simulink model "position_control"  (R2026a)
settings: Solver=VariableStepAuto  StopTime=3
model workspace (MAT data in the model file):
  K = Simulink.Parameter
  K.Complexity = 'real'
  K.Dimensions = [0 0]
  K.DataType = 'auto'
  Kp = Simulink.Parameter
  Kp.Complexity = 'real'
  Kp.Dimensions = [0 0]
  Kp.DataType = 'auto'
  omega_d = Simulink.Parameter
  omega_d.Complexity = 'real'
  omega_d.Dimensions = [0 0]
  omega_d.DataType = 'auto'
  sigma = Simulink.Parameter
  sigma.Complexity = 'real'
  sigma.Dimensions = [0 0]
  sigma.DataType = 'auto'
values from neighbouring files (symbols this model uses):
  K = 1.75    [Runpos_control.m]
  Kp = 2    [Runpos_control.m]
  sigma = 17.5    [Runpos_control.m]
libraries: simulink x1, slpidlib x1
settings Model: Creator=tmpad  LastModifiedBy=tmpad

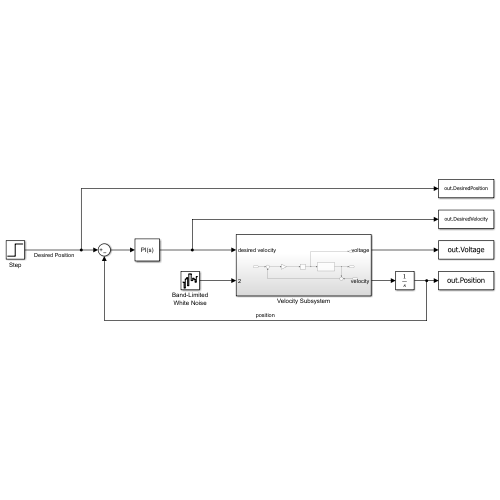
[thumbnail: Simulink's stored preview of the top-level diagram]
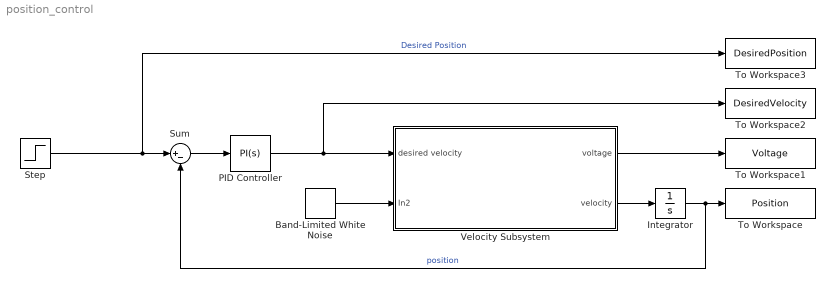
== system position_control ==
  Band-Limited White Noise : simulink/Sources/Band-Limited White Noise  Cov=[0.0001]  Ts=0.01  seed=[23341]
  Integrator : Integrator
  PID Controller : slpidlib/PID Controller  Controller=PI  Form=Parallel  TimeDomain=Continuous-time  UseExternalTs=off  SampleTime=-1  IntegratorMethod=Forward Euler  FilterMethod=Forward Euler  ControllerParametersSource=internal  P=1  I=1  UseKiTs=off  D=0  UseExternalDerivativeSource=off  N=100  UseFilter=on  TunerSelectOption=Transfer Function Based (PID Tuner App)  InitialConditionSource=internal  InitialConditionForIntegrator=0  InitialConditionForFilter=0  DifferentiatorICPrevScaledInput=0  ExternalReset=none  TrackingMode=off  Kt=1  LimitOutput=off  SatLimitsSource=internal  UpperSaturationLimit=inf  LowerSaturationLimit=-inf  LinearizeAsGain=on  AntiWindupMode=none  Kb=1  LimitIntegrator=off  UpperIntegratorSaturationLimit=inf  LowerIntegratorSaturationLimit=-inf  POutMin=[]  POutMax=[]  IOutMin=[]  IOutMax=[]  DOutMin=[]  DOutMax=[]  NOutMin=[]  NOutMax=[]  SumOutMin=[]  SumOutMax=[]  SaturationOutMin=[]  SaturationOutMax=[]  PParamMin=[]  PParamMax=[]  IParamMin=[]  IParamMax=[]  DParamMin=[]  DParamMax=[]  NParamMin=[]  NParamMax=[]  KbParamMin=[]  KbParamMax=[]  KtParamMin=[]  KtParamMax=[]  KbOutMin=[]  KbOutMax=[]  KtOutMin=[]  KtOutMax=[]  IntegratorOutMin=[]  IntegratorOutMax=[]  FilterOutMin=[]  FilterOutMax=[]  SumI1OutMin=[]  SumI1OutMax=[]  SumI2OutMin=[]  SumI2OutMax=[]  SumI3OutMin=[]  SumI3OutMax=[]  SumI4OutMin=[]  SumI4OutMax=[]  SumDOutMin=[]  SumDOutMax=[]  DifferentiatorOutMin=[]  DifferentiatorOutMax=[]  FilterDiffOutCoefMin=[]  FilterDiffOutCoefMax=[]  ReciprocalOutMin=[]  ReciprocalOutMax=[]  SumDenOutMin=[]  SumDenOutMax=[]  SumNumOutMin=[]  SumNumOutMax=[]  DivideOutMin=[]  DivideOutMax=[]  UdiffTsProdOutMin=[]  UdiffTsProdOutMax=[]  NTsProdOutMin=[]  NTsProdOutMax=[]  UintegralTsProdOutMin=[]  UintegralTsProdOutMax=[]  UngainTsProdOutMin=[]  UngainTsProdOutMax=[]  ClampingZeroOutDataTypeStr=Inherit: Inherit via back propagation  ClampingZeroOutMin=[]  ClampingZeroOutMax=[]  FilterDenConstantOutDataTypeStr=Inherit: Inherit via back propagation  FilterDenConstantOutMin=[]  FilterDenConstantOutMax=[]  PCopyOutDataTypeStr=Inherit: Inherit via back propagation  PCopyOutMin=[]  PCopyOutMax=[]  NCopyOutDataTypeStr=Inherit: Inherit via back propagation  NCopyOutMin=[]  NCopyOutMax=[]  IntegratorContinuousStateAttributes=''  IntegratorStateMustResolveToSignalObject=off  IntegratorRTWStateStorageClass=Auto  FilterContinuousStateAttributes=''  FilterStateMustResolveToSignalObject=off  FilterRTWStateStorageClass=Auto  ParallelPVariant=InternalParameters  IdealPVariant=Disabled  IVariant=InternalParameters  DVariant=Disabled  IntegratorVariant=Continuous  SatVariant=Disabled  AWVariant=Passthrough  PCopyVariant=Disabled  TRVariant=Disabled  FdbkBlocksVariant=Forward  IdealPFdbkVariant=Disabled  SatFdbkVariant=Disabled  DerivativeFilterVariant=Disabled  NVariant=Disabled  NCopyVariant=Disabled_SignalSpec  FilterICVariant=Disabled  IntegratorICVariant=InternalICs  ExternalResetVariant=Disabled  TRSumVariant=Passthrough  SumFdbkVariant=Disabled  SumVariant=Sum_PI  TsampFilterVariant=InternalTs  TsampNgainVariant=Passthrough  TsampIntegralVariant=Disabled_SignalSpec  ExternalSaturationOutDataTypeStr=Inherit: Same as second input  DerivativeSourceVariant=Disabled  PreIntVariant=InternalPreInt
  Step : Step  FinalValue=omega_d  SampleTime=0
  Sum : Sum  Inputs=|+-
  To Workspace : ToWorkspace  VariableName=Position  SaveFormat=Timeseries  SampleTime=-1
  To Workspace1 : ToWorkspace  VariableName=Voltage  SaveFormat=Timeseries  SampleTime=-1
  To Workspace2 : ToWorkspace  VariableName=DesiredVelocity  SaveFormat=Timeseries  SampleTime=-1
  To Workspace3 : ToWorkspace  VariableName=DesiredPosition  SaveFormat=Timeseries  SampleTime=-1
  Velocity Subsystem : Subsystem
  wires:
  PID Controller/1 -> To Workspace2/1, Velocity Subsystem/1(desired velocity)
  Band-Limited White Noise/1 -> Velocity Subsystem/2(In2)
  Velocity Subsystem/1(voltage) -> To Workspace1/1
  Velocity Subsystem/2(velocity) -> Integrator/1
  Sum/1 -> PID Controller/1
  Step/1 -> To Workspace3/1, Sum/1  "Desired Position"
  Integrator/1 -> Sum/2, To Workspace/1  "position"

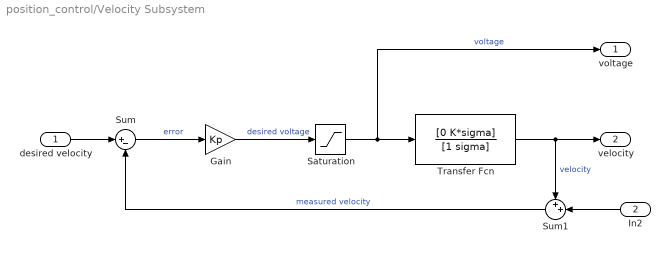
== system position_control/Velocity Subsystem ==
  desired velocity : Inport
  In2 : Inport  Port=2
  Gain : Gain  Gain=Kp
  Saturation : Saturate  UpperLimit=7.5  LowerLimit=-7.5
  Sum : Sum  Inputs=|+-
  Sum1 : Sum  Inputs=++|
  Transfer Fcn : TransferFcn  Numerator=[0 K*sigma]  Denominator=[1 sigma]
  voltage : Outport
  velocity : Outport  Port=2
  wires:
  Gain/1 -> Saturation/1  "desired voltage"
  Transfer Fcn/1 -> velocity/1, Sum1/1  "velocity"
  Saturation/1 -> voltage/1, Transfer Fcn/1  "voltage"
  Sum/1 -> Gain/1  "error"
  In2/1 -> Sum1/2
  desired velocity/1 -> Sum/1
  Sum1/1 -> Sum/2  "measured velocity"
